simulink model "Estimation"  (R2026a)
settings: Solver=FixedStepAuto  FixedStep=SIM.FixedStepSize
undefined symbols (not defined in the file): EST, MAV, SNS
settings Model: Creator=emrec  LastModifiedBy=emrec

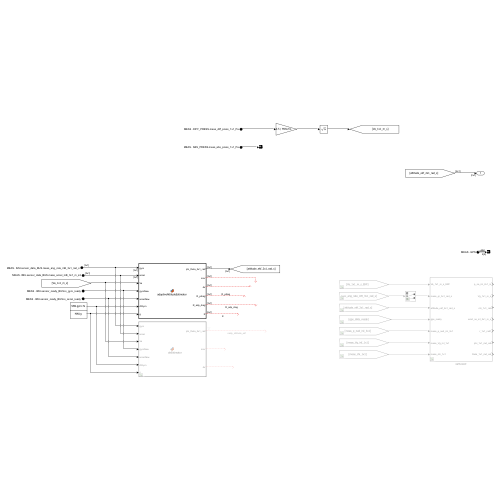
[thumbnail: Simulink's stored preview of the top-level diagram]
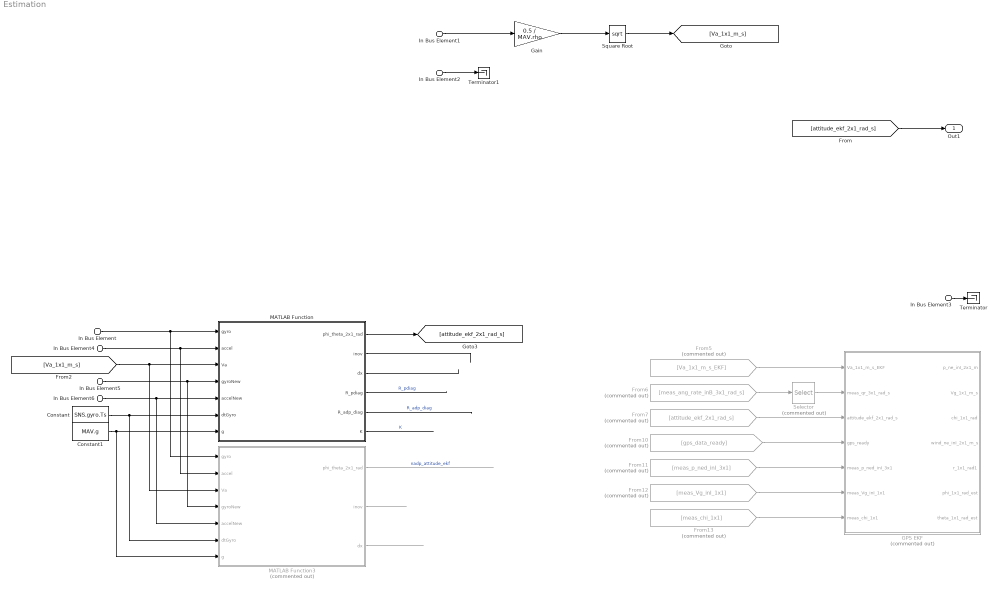
== system Estimation ==
  In Bus Element4 : Inport  PortName=MEAS  Element=IMU.sensor_data_BUS.meas_accel_inB_3x1_m_s2
  In Bus Element : Inport  PortName=MEAS  Element=IMU.sensor_data_BUS.meas_ang_rate_inB_3x1_rad_s
  In Bus Element6 : Inport  PortName=MEAS  Element=IMU.sensor_ready_BUS.is_accel_ready
  In Bus Element5 : Inport  PortName=MEAS  Element=IMU.sensor_ready_BUS.is_gyro_ready
  In Bus Element2 : Inport  PortName=MEAS  Element=ABS_PRESS.meas_abs_press_1x1_Pa
  In Bus Element1 : Inport  PortName=MEAS  Element=DIFF_PRESS.meas_diff_press_1x1_Pa
  In Bus Element3 : Inport  PortName=MEAS  Element=GPS
  Constant : Constant  Value=SNS.gyro.Ts
  Constant1 : Constant  Value=MAV.g
  From10 : From  Commented=on  GotoTag=gps_data_ready
  From11 : From  Commented=on  GotoTag=meas_p_ned_inI_3x1
  From12 : From  Commented=on  GotoTag=meas_Vg_inI_1x1
  From13 : From  Commented=on  GotoTag=meas_chi_1x1
  From5 : From  Commented=on  GotoTag=Va_1x1_m_s_EKF
  From6 : From  Commented=on  GotoTag=meas_ang_rate_inB_3x1_rad_s
  From7 : From  Commented=on  GotoTag=attitude_ekf_2x1_rad_s
  GPS EKF : Subsystem  Commented=on
  Gain : Gain  Gain=0.5 / MAV.rho
  MATLAB Function : MATLAB Function  TreatAsAtomicUnit=on  SystemSampleTime=EST.SamplingTime
  MATLAB Function3 : MATLAB Function  Commented=on  TreatAsAtomicUnit=on  SystemSampleTime=EST.SamplingTime
  Selector : Selector  Commented=on  InputPortWidth=3  IndexOptions=Index vector (dialog)  Indices=[2 3]  OutputSizes=1
  Square Root : Sqrt
  Terminator : Terminator
  Terminator1 : Terminator
  Out1 : Outport
  wires:
  From13/1 -> GPS EKF/7(meas_chi_1x1)
  From12/1 -> GPS EKF/6(meas_Vg_inI_1x1)
  From11/1 -> GPS EKF/5(meas_p_ned_inI_3x1)
  From10/1 -> GPS EKF/4(gps_ready)
  From7/1 -> GPS EKF/3(attitude_ekf_2x1_rad_s)
  MATLAB Function/1(phi_theta_2x1_rad) -> [attitude_ekf_2x1_rad_s]
  Selector/1 -> GPS EKF/2(meas_qr_3x1_rad_s)
  From6/1 -> Selector/1
  From5/1 -> GPS EKF/1(Va_1x1_m_s_EKF)
  [Va_1x1_m_s] -> MATLAB Function3/3(Va), MATLAB Function/3(Va)
  Square Root/1 -> [Va_1x1_m_s]
  Gain/1 -> Square Root/1
  In Bus Element1/1 -> Gain/1
  In Bus Element3/1 -> Terminator/1
  In Bus Element2/1 -> Terminator1/1
  [attitude_ekf_2x1_rad_s] -> Out1/1
  In Bus Element/1 -> MATLAB Function3/1(gyro), MATLAB Function/1(gyro)
  In Bus Element5/1 -> MATLAB Function3/4(gyroNew), MATLAB Function/4(gyroNew)
  In Bus Element4/1 -> MATLAB Function3/2(accel), MATLAB Function/2(accel)
  In Bus Element6/1 -> MATLAB Function3/5(accelNew), MATLAB Function/5(accelNew)
  Constant/1 -> MATLAB Function3/6(dtGyro), MATLAB Function/6(dtGyro)
  Constant1/1 -> MATLAB Function3/7(g), MATLAB Function/7(g)
  MATLAB Function/2(inov) -> ?
  MATLAB Function/3(dx) -> ?
  MATLAB Function/4(R_pdiag) -> ?  "R_pdiag"
  MATLAB Function/5(R_adp_diag) -> ?  "R_adp_diag"
  MATLAB Function/6(K) -> ?  "K"
  MATLAB Function3/1(phi_theta_2x1_rad) -> ?  "nadp_attitude_ekf"
  MATLAB Function3/3(dx) -> ?
  MATLAB Function3/2(inov) -> ?

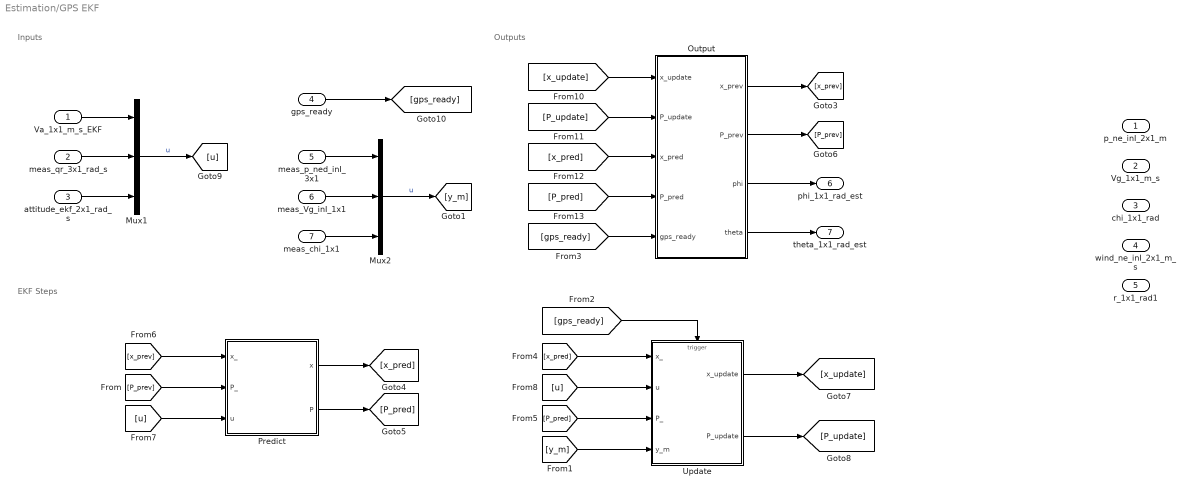
== system Estimation/GPS EKF ==
  note: EKF Steps
  note: Outputs
  note: Inputs
  Va_1x1_m_s_EKF : Inport
  meas_qr_3x1_rad_s : Inport  Port=2
  attitude_ekf_2x1_rad_s : Inport  Port=3
  gps_ready : Inport  Port=4
  meas_p_ned_inI_3x1 : Inport  Port=5
  meas_Vg_inI_1x1 : Inport  Port=6
  meas_chi_1x1 : Inport  Port=7
  Mux1 : Mux  Inputs=3
  Mux2 : Mux  Inputs=3
  Output : Subsystem  TreatAsAtomicUnit=on
  Predict : Subsystem
  Update : Subsystem  TreatAsAtomicUnit=on
  p_ne_inI_2x1_m : Outport
  Vg_1x1_m_s : Outport  Port=2
  chi_1x1_rad : Outport  Port=3
  wind_ne_inI_2x1_m_s : Outport  Port=4
  r_1x1_rad1 : Outport  Port=5
  phi_1x1_rad_est : Outport  Port=6
  theta_1x1_rad_est : Outport  Port=7
  wires:
  Mux2/1 -> [y_m]  "u"
  meas_p_ned_inI_3x1/1 -> Mux2/1
  meas_Vg_inI_1x1/1 -> Mux2/2
  meas_chi_1x1/1 -> Mux2/3
  gps_ready/1 -> [gps_ready]
  Mux1/1 -> [u]  "u"
  attitude_ekf_2x1_rad_s/1 -> Mux1/3
  meas_qr_3x1_rad_s/1 -> Mux1/2
  Va_1x1_m_s_EKF/1 -> Mux1/1
  [x_pred] -> Update/1(x_)
  Update/2(P_update) -> [P_update]
  [P_pred] -> Update/3(P_)
  [gps_ready] -> Update/Trigger
  Output/4(theta) -> theta_1x1_rad_est/1
  [u] -> Update/2(u)
  [x_update] -> Output/1(x_update)
  Output/3(phi) -> phi_1x1_rad_est/1
  [P_prev] -> Predict/2(P_)
  [gps_ready] -> Output/5(gps_ready)
  [y_m] -> Update/4(y_m)
  [x_prev] -> Predict/1(x_)
  [P_pred] -> Output/4(P_pred)
  Update/1(x_update) -> [x_update]
  Predict/1(x) -> [x_pred]
  Output/1(x_prev) -> [x_prev]
  [u] -> Predict/3(u)
  Predict/2(P) -> [P_pred]
  [x_pred] -> Output/3(x_pred)
  Output/2(P_prev) -> [P_prev]
  [P_update] -> Output/2(P_update)

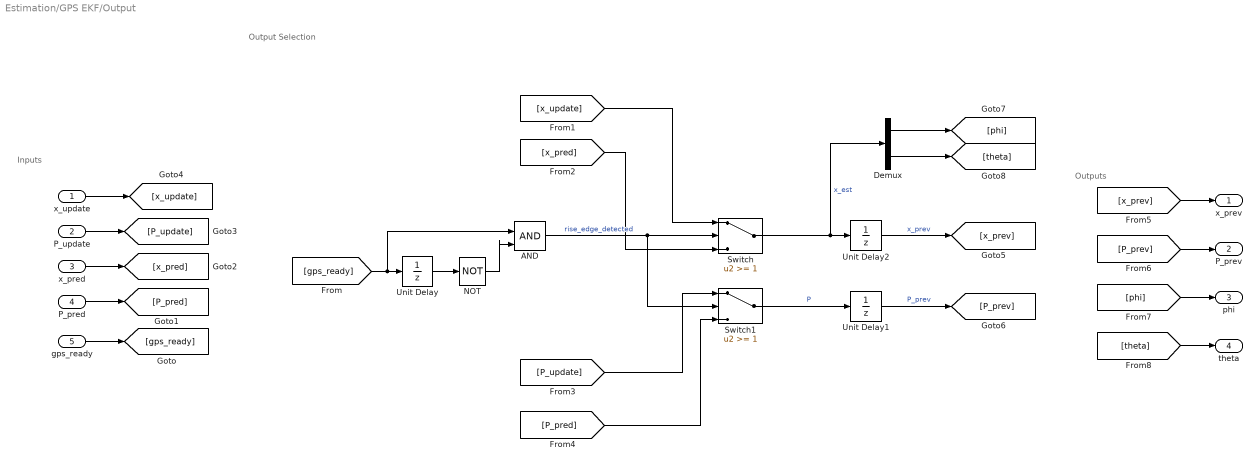
== system Estimation/GPS EKF/Output ==
  note: Inputs
  note: Outputs
  note: Output Selection
  x_update : Inport
  P_update : Inport  Port=2
  x_pred : Inport  Port=3
  P_pred : Inport  Port=4
  gps_ready : Inport  Port=5
  AND : Logic  IconShape=distinctive  AllPortsSameDT=off  OutDataTypeStr=boolean
  Demux : Demux  Outputs=2
  NOT : Logic  Operator=NOT  IconShape=distinctive  AllPortsSameDT=off  OutDataTypeStr=boolean
  Switch : Switch  Threshold=1  SaturateOnIntegerOverflow=off  InputSameDT=off
  Switch1 : Switch  Threshold=1  SaturateOnIntegerOverflow=off  InputSameDT=off
  Unit Delay : UnitDelay  SampleTime=-1
  Unit Delay1 : UnitDelay  InitialCondition=EST.attitude_ekf.init_P  SampleTime=-1
  Unit Delay2 : UnitDelay  InitialCondition=EST.attitude_ekf.init_states  SampleTime=-1
  x_prev : Outport
  P_prev : Outport  Port=2
  phi : Outport  Port=3
  theta : Outport  Port=4
  wires:
  [theta] -> theta/1
  [phi] -> phi/1
  Demux/1 -> [phi]
  Demux/2 -> [theta]
  [P_prev] -> P_prev/1
  [x_prev] -> x_prev/1
  Unit Delay2/1 -> [x_prev]  "x_prev"
  Unit Delay1/1 -> [P_prev]  "P_prev"
  Switch1/1 -> Unit Delay1/1  "P"
  Switch/1 -> Unit Delay2/1, Demux/1  "x_est"
  [P_pred] -> Switch1/3
  [P_update] -> Switch1/1
  [x_pred] -> Switch/3
  [x_update] -> Switch/1
  [gps_ready] -> Unit Delay/1, AND/1
  x_update/1 -> [x_update]
  P_update/1 -> [P_update]
  x_pred/1 -> [x_pred]
  P_pred/1 -> [P_pred]
  gps_ready/1 -> [gps_ready]
  AND/1 -> Switch/2, Switch1/2  "rise_edge_detected"
  NOT/1 -> AND/2
  Unit Delay/1 -> NOT/1

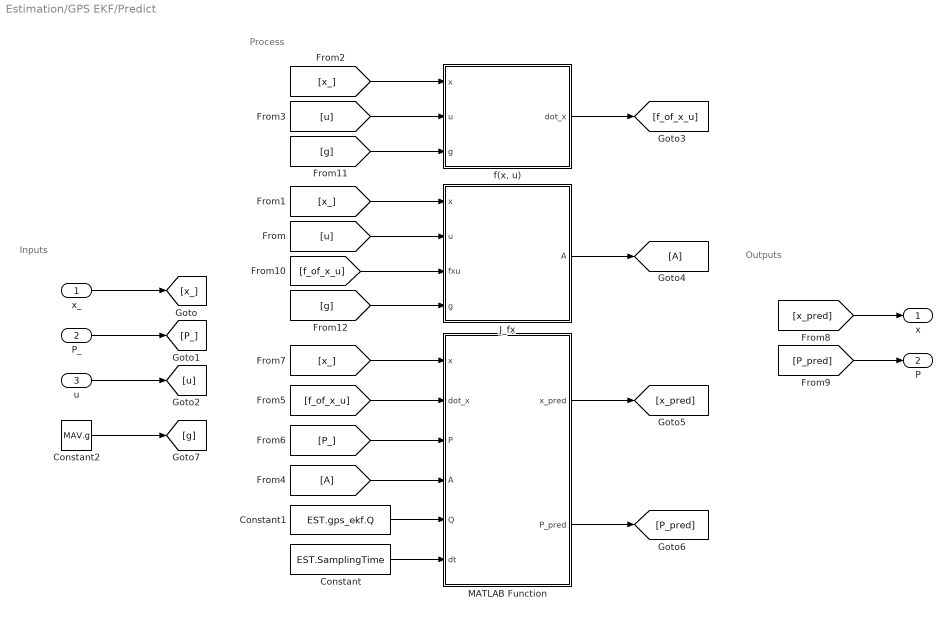
== system Estimation/GPS EKF/Predict ==
  note: Inputs
  note: Outputs
  note: Process
  x_ : Inport
  P_ : Inport  Port=2
  u : Inport  Port=3
  Constant : Constant  Value=EST.SamplingTime
  Constant1 : Constant  Value=EST.gps_ekf.Q
  Constant2 : Constant  Value=MAV.g
  From4 : From
  Goto4 : Goto
  J_fx : MATLAB Function  TreatAsAtomicUnit=on
  MATLAB Function : MATLAB Function  TreatAsAtomicUnit=on
  "f(x, u)" : MATLAB Function  TreatAsAtomicUnit=on
  x : Outport
  P : Outport  Port=2
  wires:
  [g] -> J_fx/4(g)
  [g] -> "f(x, u)"/3(g)
  Constant2/1 -> [g]
  [f_of_x_u] -> J_fx/3(fxu)
  [P_pred] -> P/1
  [x_pred] -> x/1
  MATLAB Function/2(P_pred) -> [P_pred]
  MATLAB Function/1(x_pred) -> [x_pred]
  [x_] -> MATLAB Function/1(x)
  [P_] -> MATLAB Function/3(P)
  [f_of_x_u] -> MATLAB Function/2(dot_x)
  From4/1 -> MATLAB Function/4(A)
  J_fx/1(A) -> Goto4/1
  "f(x, u)"/1(dot_x) -> [f_of_x_u]
  [u] -> "f(x, u)"/2(u)
  [x_] -> "f(x, u)"/1(x)
  [x_] -> J_fx/1(x)
  [u] -> J_fx/2(u)
  Constant1/1 -> MATLAB Function/5(Q)
  Constant/1 -> MATLAB Function/6(dt)
  u/1 -> [u]
  P_/1 -> [P_]
  x_/1 -> [x_]

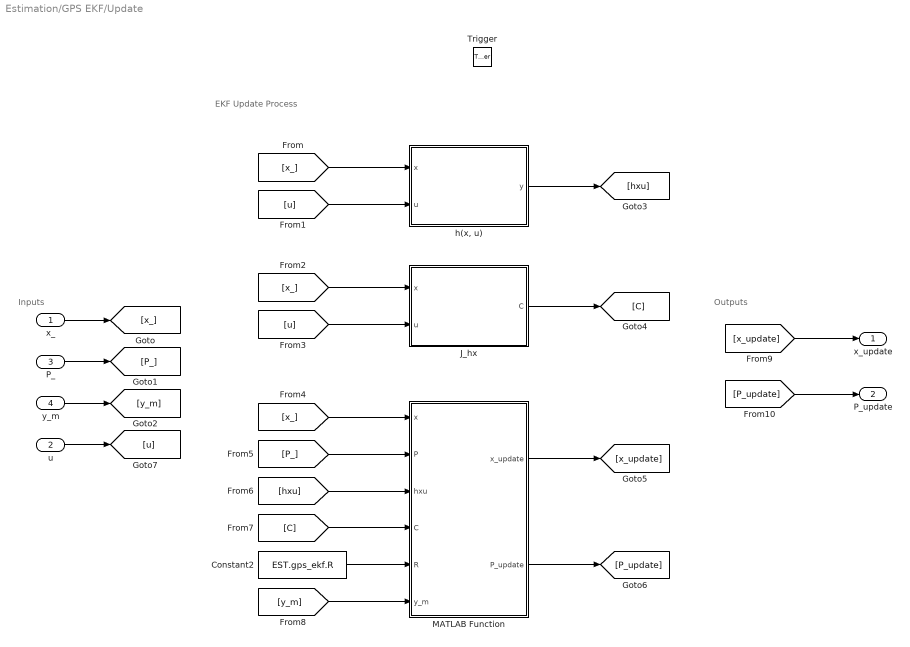
== system Estimation/GPS EKF/Update ==
  note: Inputs
  note: EKF Update Process
  note: Outputs
  x_ : Inport
  u : Inport  Port=2
  P_ : Inport  Port=3
  y_m : Inport  Port=4
  Trigger : TriggerPort  VariantControl=(inherit)  PortDimensions=1
  Constant2 : Constant  Value=EST.gps_ekf.R
  J_hx : MATLAB Function  TreatAsAtomicUnit=on
  MATLAB Function : MATLAB Function  TreatAsAtomicUnit=on
  "h(x, u)" : MATLAB Function  TreatAsAtomicUnit=on
  x_update : Outport
  P_update : Outport  Port=2
  wires:
  u/1 -> [u]
  [x_update] -> x_update/1
  [P_update] -> P_update/1
  MATLAB Function/2(P_update) -> [P_update]
  MATLAB Function/1(x_update) -> [x_update]
  [y_m] -> MATLAB Function/6(y_m)
  Constant2/1 -> MATLAB Function/5(R)
  [C] -> MATLAB Function/4(C)
  J_hx/1(C) -> [C]
  [hxu] -> MATLAB Function/3(hxu)
  "h(x, u)"/1(y) -> [hxu]
  [P_] -> MATLAB Function/2(P)
  [x_] -> MATLAB Function/1(x)
  [x_] -> J_hx/1(x)
  [u] -> J_hx/2(u)
  [u] -> "h(x, u)"/2(u)
  [x_] -> "h(x, u)"/1(x)
  y_m/1 -> [y_m]
  P_/1 -> [P_]
  x_/1 -> [x_]

== matlab function Estimation/GPS EKF/Update/h(x, u) ==
  data: x input; u input; y output
function y = output_equation(x, u)
    y = zeros(6, 1);
    y(1:4) = x(1:4);
    
    c_psi = cos(x(7));
    s_psi = sin(x(7));

    c_chi = cos(x(4));
    s_chi = sin(x(4));

    y(5) = u(1)* c_psi + x(5) - x(3) * c_chi;
    y(6) = u(1) * s_psi + x(6) - x(3) * s_chi;
end

== matlab function Estimation/MATLAB Function ==
  data: gyro input; accel input; Va input; gyroNew input; accelNew input; dtGyro input; phi_theta_2x1_rad output; g input; EST parameter; inov output; dx output; R_pdiag output; R_adp_diag output; K output
function [phi_theta_2x1_rad, inov, dx, R_pdiag, R_adp_diag, K] = adaptiveAttitudeEstimator(gyro, accel, Va, gyroNew, accelNew, dtGyro, g, EST)

    persistent attEst
    EST_ = EST.attitude_ekf;

    if isempty(attEst)

        attEst = AdaptiveAttitudeEstimator(EST_.init_states, EST_.init_P, ...
                                   EST_.Q, EST_.R, g, EST_.gamma, EST_.alpha, EST_.beta, EST_.R_max);
    end

    [phi_theta_2x1_rad, ~, inov, ~, dx] = attEst.step(gyro, accel, Va, gyroNew, accelNew, dtGyro);

    R_pdiag = diag(attEst.diagnostics.R_prev);
    R_adp_diag = diag(attEst.diagnostics.R_adp);
    K = attEst.diagnostics.K(:);
end

== matlab function Estimation/MATLAB Function3 ==
  data: gyro input; accel input; Va input; gyroNew input; accelNew input; dtGyro input; phi_theta_2x1_rad output; g input; EST parameter; inov output; dx output
function [phi_theta_2x1_rad, inov, dx] = attitudeEstimator(gyro, accel, Va, gyroNew, accelNew, dtGyro, g, EST)
    persistent attEst
    EST_ = EST.attitude_ekf;

    if isempty(attEst)
        attEst = AttitudeEstimator(EST_.init_states, EST_.init_P, ...
                                   EST_.Q, EST_.R, g);
    end

    [phi_theta_2x1_rad, ~, inov, ~, dx] = attEst.step(gyro, accel, Va, gyroNew, accelNew, dtGyro);


end

== matlab function Estimation/GPS EKF/Predict/J_fx ==
  data: x input; u input; A output; fxu input; g input
function A = Jacobian_fx(x, u, fxu, g)
    A = zeros(7,7); 

    c_chi = cos(x(4));
    s_chi = sin(x(4));

    s_phi = sin(u(4));
    c_phi = cos(u(4));
    t_phi = s_phi / c_phi;

    s_theta = sin(u(5));
    c_theta = cos(u(5));

    c_chi_mpsi = cos(x(4) - x(7));
    s_chi_mpsi = sin(x(4) - x(7));
    c_psi = cos(x(7));
    s_psi = sin(x(7));

    % pd f / pd x(3), x(3) = Vg
    A(1, 3) = c_chi;
    A(2, 3) = s_chi;
    A(3, 3) = - fxu(3) / x(3);
    A(4, 3) = - fxu(4) / x(3);

    % pd f / pd x(4), x(4) = chi
    A(1, 4) = -x(3) * s_chi;
    A(2, 4) = x(3) * c_chi;
    A(4, 4) = g * t_phi / x(3) * (-s_chi_mpsi);

    % pdf / pdx(5), x(5) = wn
    A(3, 5) = -fxu(7) * u(1) * s_psi / x(3); 
    
    % pdf / pdx(6), x(6) = we
    A(3, 6) = fxu(7) * u(1) * c_psi / x(3); 

    % pdf / pdx(6), x(7) = psi
    A(3, 7) = 1 / x(3) * (-fxu(7) * u(1)) * (x(5)*c_psi + x(6)*s_psi);
    A(4, 7) = g / x(3) * t_phi * s_chi_mpsi;
end

== matlab function Estimation/GPS EKF/Predict/MATLAB Function ==
  data: x input; dot_x input; x_pred output; P input; A input; Q input; dt input; P_pred output
function [x_pred, P_pred] = ekf_predict_step(x, dot_x, P, A, Q, dt)
    % Propagation with Euler Numerical Integration
    x_pred = x + dt * dot_x;
    P_pred = P + (A*P + P*A'+ Q) * dt;
    P_pred = 0.5 * (P_pred + P_pred');
end

== matlab function Estimation/GPS EKF/Predict/f(x, u) ==
  data: x input; u input; dot_x output; g input
function dot_x = state_equation(x, u, g)
    dot_x = zeros(7,1);

    c_chi = cos(x(4));
    s_chi = sin(x(4));

    s_phi = sin(u(4));
    c_phi = cos(u(4));
    t_phi = s_phi / c_phi;

    % s_theta = sin(u(5));
    c_theta = cos(u(5));

    c_chi_mpsi = cos(x(4) - x(7));
    c_psi = cos(x(7));
    s_psi = sin(x(7));

    dot_psi = u(2) * s_phi / c_theta + u(3)* c_phi / c_theta;

    dot_x(1) = x(3) * c_chi;
    dot_x(2) = x(3) * s_chi;
    dot_x(4) = g / x(3) * c_chi_mpsi * t_phi;

    dot_x(5:6) = zeros(2, 1);

    num = (u(1) * c_psi + x(5)) * (- u(1) *dot_psi * s_psi) ...
        + (u(1)* s_psi + x(6)) * (u(1)*dot_psi * c_psi);

    dot_x(3) = num / x(3);

    dot_x(7) = dot_psi;


end

== matlab function Estimation/GPS EKF/Update/J_hx ==
  data: x input; u input; C output
function C = Jacobian_hx(x, u)
    C = zeros(6, 7);
    C(1:4, 1:4) = eye(4, 4);
    
    C(5, 3) = -cos(x(4));
    C(6, 3) = -sin(x(4));

    C(5, 4) = x(3) * sin(x(4));
    C(6, 4) = - x(3) * cos(x(4));

    C(5, 5) = 1;
    C(6, 6) = 1;

    C(5, 7) = -u(1) * sin(x(7));
    C(6, 7) = u(1) * cos(x(7));
end

== matlab function Estimation/GPS EKF/Update/MATLAB Function ==
  data: x input; x_update output; P input; hxu input; C input; R input; y_m input; P_update output
function [x_update, P_update] = ekf_update_step(x, P, hxu, C, R, y_m)
    S = C*P*C' + R;
    L = P*C' / S;
    
    % shape = size(P);
    shape = [7, 7]; 
    P_update = (eye(shape) - L * C)*P;
    x_update = x + L * (y_m - hxu);
    P_update = 0.5 * (P_update + P_update');
end
